simulink model "vrm_plus_ff_return_backup"  (R2013a)
settings: Solver=ode4  SolverMode=SingleTasking  StartTime=0.0  StopTime=inf  FixedStep=0.0005  RelTol=1e-3
StartFcn:
  |  warndlg('Dexterit-E models cannot run under simulation. Please compile your model and run it from within Dexterit-E.');set_param(bdroot,'SimulationCommand','stop')
model workspace (MAT data in the model file):
  BKIN_STEP_TIME = 0.0005
  col_x = 1
  col_y = 2
  E_TARGET_ON = 3
  E_HOLD_AT_TARGET = 5
  LOGICAL_RADIUS = 4
  START_TARGET_COL = 1
  END_TARGET_COL = 2
  ROTATION_CENTER = 3
  WAIT_AT_1stTARGET_COL = 4
  MAXREACHTIME_COL = 5
  WAIT_AT_2ndTARGET_COL = 6
  ROTATION_TYPE = 8
  ROTATION = 9
  DELAY_POSTTRIAL_COL = 7
  E_STAY_CENTER = 2
  VISUAL_RADIUS = 3
  COLOR = 5
  ALTCOLOR = 6
  A_VISC = 1
  B_VISC = 2
  C_VISC = 3
  D_VISC = 4
  LOAD = 10
  TRAJ_DURATION_COL = 11
undefined symbols (not defined in the file or in its folder): slselsubs
libraries: General x3, KINARM_EP_loads x3, Video x3, KINARM_general x1, simulink x1, KINARM_loads x1
(part 1 of 2)
CloseFcn:
  | rtwprivate ssgencode ModelCloseRequest b2lab2d
settings Model: ModifiedComment=chris -- Wed Feb 16 09:18:30 2005 -- Version 1.1384  ModifiedHistory=Feb 16/05 - Add error repeat, add offset ramp  ExtModeArmWhenConnect=off  ExtModeLogAll=off  BufferReuse=off  Creator=Chris Grebeldinger  LastModifiedBy=BKIN TECHNOLOGIES
settings DataIOCC: LimitDataPoints=off  SignalLoggingSaveFormat=ModelDataLogs  SaveOutput=off  SaveTime=off  SignalLoggingName=sigsOut
settings OptimizationCC: BlockReduction=off  BooleanDataType=off  OptimizeBlockIOStorage=off  BufferReuse=off  ExpressionFolding=off  ExpressionDepthLimit=2147483647  FoldNonRolledExpr=off  LocalBlockOutputs=off  InitFltsAndDblsToZero=on
settings DebuggingCC: SaveWithParameterizedLinksMsg=none  SignalResolutionControl=TryResolveAllWithWarning  SolverPrmCheckMsg=none  MultiTaskDSMMsg=warning  MultiTaskCondExecSysMsg=none  FcnCallInpInsideContextMsg=UseLocalSettings  StrictBusMsg=None
settings HardwareCC: ProdIntDivRoundTo=Zero  ProdEndianess=LittleEndian  ProdHWDeviceType=Generic->32-bit x86 compatible  TargetHWDeviceType=32-bit Generic
settings SFSimCC: SimParseCustomCode=off
settings RTWCC: SystemTargetFile=xpctarget.tlc  TemplateMakefile=xpc_default_tmf  Description=xPC Target  ProcessScript=xpctarget_make_rtw_hook  IncludeERTFirstTime=on  RTWCompilerOptimization=On
settings CodeAppCC: MaxIdLength=63
settings xpcTargetCC: TargetFcnLib=ansi_tfl_tmw.mat  CodeReplacementLibrary=XPC_BLAS  ParMdlRefBuildCompliant=on  ConcurrentExecutionCompliant=on  CombineSignalStateStructs=off  MATLABClassNameForMDSCustomization=xpcAperiodicCustomization  GRTInterface=on  GenerateAllocFcn=off  xPCTaskExecutionProfile=off  xPCRL32EventNumber=5000  xPCisDownloadable=off  xPCLoadParamSetFile=off  xPCConcurrentTasks=off  xPCEnableSFAnimation=off

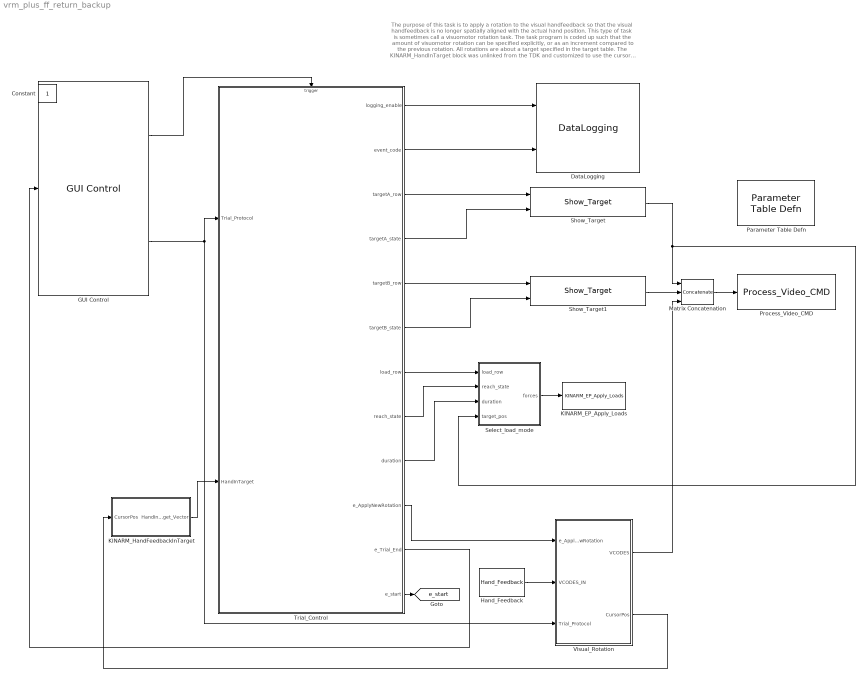
== system vrm_plus_ff_return_backup ==
  note: The purpose of this task is to apply a rotation to the visual handfeedback so that the visual handfeedback is no longer spatially aligned with the actual hand position.
      | This type of task is sometimes call a visuomotor rotation task.
      | The task program is coded up such that the amount of visuomotor rotation can be specified explicitly, or as an increment compared to the previous rotation.
      | All rotations are about a target specified in the target table.
      |
      | The KINARM_HandInTarget block was unlinked from the TDK and customized to use the cursor position as hand feedback input, rather than the KINARM robot's actual location.
  DataLogging : General/DataLogging  log_event_codes=on  log_analog_inputs=off
      link override Poll KINARM/EPTorqueCMD: GotoTag=KINARMEPTorqueCMD
  GUI Control : General/GUI Control  target_type_str=Circle  Target_Type=1  XYcols=[1 2]  Vcols=3  Lcols=4  indices_padding=[0 0 0 0;0 0 0 0]  task_version=1.0  show_repeat_trial_flag=off
  Hand_Feedback : KINARM_general/Hand_Feedback  feedback_cntl_src=none
  KINARM_EP_Apply_Loads : KINARM_EP_loads/KINARM_EP_Apply_Loads  up_duration=1500  down_duration=1500  max_force=60
  KINARM_HandFeedbackInTarget : Subsystem  AncestorBlock=KINARM_general/KINARM_HandInTarget  mask(KINARM_HandInTarget){use_dominant_hand=on, target_type=Circle, num_states=1, attribcol1=4, attribcol2=3, attribcol3=3, attribcol4=3}
      mask prompts: use_dominant_hand "Dominant Hand?"; target_type "Type of Target"; num_states "Number of Target States"; attribcol1 "State 1 Target Table Column(s)"; attribcol2 "State 2 Target Table Column(s)"; attribcol3 "State 3 Target Table Column(s)"; attribcol4 "State 4 Target Table Column(s)"
      mask help: This block returns a vector or array corresponding to the Target_Table rows indicating whether the specified hand is in (=1) or out (=0) of each of the targets.
      mask init:
      | num_states=str2num(get_param(gcb, 'num_states'));
      | columntext='(columns: ';
      | 
      | for i=1:num_states
      | 	varname=['attribcol' num2str(i)];
      | 	if i>1
      | 		columntext=[columntext, '; '];
      | 	end
      | 	columntext=[columntext, get_param(gcb, varname)];
      | end
      | columntext=strvcat([columntext ')'],' ', ' ');
      | 
      | output_block=char(find_system(gcb,'LookUnderMasks','all','FollowLinks','on','SearchDepth',1,'BlockType','Outport'));
      | outputname=get_param(output_block,'Name');
      | 
      | % Select only the desired states for output. The output port is also renamed to reflect 
      | % whether the output is a vector (in the case of a single state) or an array (of vectors, 
      | % one for each of multiple states).
      | if num_states == 1
      | 	set_param([gcb '/Selected States'], 'Value', '[1]');
      | 	set_param(output_block, 'Name', 'HandInTarget_Vector');
      | elseif num_states == 2
      | 	set_param([gcb '/Selected States'], 'Value', '[1,2]');
      | 	set_param(output_block, 'Name', 'HandInTarget_Array');
      | elseif num_states == 3
      | 	set_param([gcb '/Selected States'], 'Value', '[1,2,3]');
      | 	set_param(output_block, 'Name', 'HandInTarget_Array');
      | else
      | 	set_param([gcb '/Selected States'], 'Value', '[1,2,3,4]');
      | 	set_param(output_block, 'Name', 'HandInTarget_Array');
      | end
      mask Help:
      | Used to determine if the hand (finger-tip) is in any of the targets in the Target_Table.
      | <P>
      | <B><I>Use of this block requires that the DataLogging block (General library) be set to log KINARM data.</I></B>
      | 
      | <H2>Library </H2>
      | KINARM_general (sub-library)
      | 
      | <H2>Description </H2>
      | This block returns a vector or array corresponding to the Target_Table rows indicating whether the specified hand (i.e. finger-tip) is in or out of each of the targets.  Each element in the output vector or output array will be either a 0 (hand not in target) or a 1 (hand in target).
      | <P>
      | A vector is returned if only one target state is specified in each target row (see Parameters and Dialog Box), with each index of the vector corresponding to a row in the target table.  An array is returned if more than one target state is specified in a target row, with each row of the array corresponding to a target row and each column corresponding to the nth target state specified in each target row.
      | <P>
      | The output vector or array is typically used by a stateflow chart to affect behavior of the system.  Because this block returns hand-in-target information for all targets in the target table, multiple targets can be monitored at once (i.e. the stateflow chart could have certain transitions that occur if the hand is in one target and other transitions if it is in a different target).  Likewise, because this block returns hand-in-target information for multiple states of a single target, those multiple states can be monitored simultaneously.
      | <P>
      | Because the KINARM_HandInTarget block returns information for only one hand, two copies of this block are required if information for both hands is desired.
      | <P>
      | 
      | <H2>Parameters and Dialog Box</H2>
      | <B>Dominant Hand?:</B> this box determines which hand is used by this block : dominant hand position (checked box) or the non-dominant hand position (unchecked box).  (Note: if the end-user wants to know about both the dominant hand and the non-dominant hand, then 2 separate copies of this block are requried, one for each hand.)
      | <P>
      | <B>Type of Target:</B> Enter the type of target specified in the target table:
      | <P>
      | <B>Number of Target States:</B> Enter the number of target states specified in each target row.  Up to four target states are allowed per target row.
      | <P>
      | <B>State <n> Target Table Columns:</B> Enter the columns in the Target Table that specify the relevant target attributes.  Do this for each target state.
      | For a circle, enter the columns corresponding to logical radius (e.g. 4)
      | <BR>For an ellipse, enter the columns corresponding to major radius, minor radius, rotation angle (e.g. [4, 5, 6]).
      | <BR>For a rectangle, enter the columns corresponding to length, height, and rotation angle (e.g. [4, 5, 6]).
      | <BR>For a line, enter the columns corresponding to stroke width, endpoint in x, and endpoint in y (e.g. [3, 4, 5]).
      | <BR>For a triangle, enter the columns corresponding to length, height, peak offset, and rotation angle (e.g. [4, 5, 6, 7]).
      | 
      | <H2>Examples</H2>
      | <B>Example 1.</B>  Suppose a target row will be used to define 1 state for a circle type target and the radius of the visual target is the same radius to be used for determination of hand-in-target.  The related Target Table column is: column 6 = radius.  For this example, "State 1 Target Table Columns" would equal [6].
      | <P>
      | 
      | <B>Example 2.</B>  Suppose a target row will be used to define 1 state for a circle type target, but the radius of the visual target will be different than the radius to be used for determination of hand-in-target.  This option allows independent control over the size of the visual target versus the accuracy needed to be considered "in the target".  The related Target Table columns are: column 6 = radius1 (i.e. radius to target to be drawn); column 7 = radius2 (i.e. radius to be used for hand-in-target) .  For this example, "State 1 Target Table Columns" would equal [7].
      | <P>
      | <B>Example 3.</B>  Suppose a target row will be used to define 2 states for a circle type target, where the radius of the visual target will be a constant, but depending on the state of the system, one of 2 other and different radii will be used for determination of hand-in-target.  The related Target Table columns are: column 6 = radius1 (i.e. radius to target to be drawn); column 7 = radius2 (i.e. radius to be used for hand-in-target for state 1); column 8 = radius3 (i.e. radius to be used for hand-in-target for state 2).  For this example, "State 1 Target Table Columns" would equal [7], while "State 2 Target Table Columns" would equal [8].
      | <P>
      | 
      | <H2>Related Blocks </H2>
      | DataLogging
      mask TypeOptions target_type: Circle | Ellipse | Rectangle | Line | Triangle
      mask Callback target_type:
      | target_type=get_param(gcb, 'target_type');
      | attribcol1=[str2num(get_param(gcb, 'attribcol1')) 0 0 0 0 0 0];
      | attribcol2=[str2num(get_param(gcb, 'attribcol2')) 0 0 0 0 0 0];
      | attribcol3=[str2num(get_param(gcb, 'attribcol3')) 0 0 0 0 0 0];
      | attribcol4=[str2num(get_param(gcb, 'attribcol4')) 0 0 0 0 0 0];
      | switch target_type(1:3)
      | 	case 'Cir'
      | 		numcol=1;
      | 	case 'Ell'
      | 		numcol=3;
      |     case 'Rec'
      |         numcol=3;
      |     case 'Lin'
      |         numcol=3;
      |     case 'Tri'
      |         numcol=4;
      | 	otherwise
      | 		numcol=1;
      | end
      | if numcol==1
      | 	set_param(gcb, 'attribcol1', num2str(attribcol1(1)));
      | 	set_param(gcb, 'attribcol2', num2str(attribcol2(1)));
      | 	set_param(gcb, 'attribcol3', num2str(attribcol3(1)));
      | 	set_param(gcb, 'attribcol4', num2str(attribcol4(1)));
      | else
      | 	set_param(gcb, 'attribcol1', ['[' num2str(attribcol1(1:numcol)) ']']);
      | 	set_param(gcb, 'attribcol2', ['[' num2str(attribcol2(1:numcol)) ']']);
      | 	set_param(gcb, 'attribcol3', ['[' num2str(attribcol3(1:numcol)) ']']);
      | 	set_param(gcb, 'attribcol4', ['[' num2str(attribcol4(1:numcol)) ']']);
      | end
      mask TypeOptions num_states: 1 | 2 | 3 | 4
      mask Callback num_states:
      | num_states = str2num(get_param(gcb, 'num_states'));
      | vis = get_param(gcb, 'MaskVisibilities');
      | 
      | % Select only the desired states for output. The output port is also renamed to reflect
      | % whether the output is a vector (in the case of a single state) or an array (of vectors,
      | % one for each of multiple states).
      | output_block=char(find_system(gcb, 'LookUnderMasks', 'all', 'FollowLinks', 'on', 'SearchDepth', 1, 'BlockType', 'Outport'));
      | 
      | if num_states == 1
      | 	set_param([gcb '/Selected States'], 'Value', '[1]');
      | 	set_param(output_block, 'Name', 'HandInTarget_Vector');
      | 	vis{5} = 'off';
      | 	vis{6} = 'off';
      | 	vis{7} = 'off';
      | elseif num_states == 2
      | 	set_param([gcb '/Selected States'], 'Value', '[1,2]');
      | 	set_param(output_block, 'Name', 'HandInTarget_Array');
      | 	vis{5} = 'on';
      | 	vis{6} = 'off';
      | 	vis{7} = 'off';
      | elseif num_states == 3
      | 	set_param([gcb '/Selected States'], 'Value', '[1,2,3]');
      | 	set_param(output_block, 'Name','HandInTarget_Array');
      | 	vis{5} = 'on';
      | 	vis{6} = 'on';
      | 	vis{7} = 'off';
      | else
      | 	set_param([gcb '/Selected States'], 'Value', '[1,2,3,4]');
      | 	set_param(output_block, 'Name', 'HandInTarget_Array');
      | 	vis{5} = 'on';
      | 	vis{6} = 'on';
      | 	vis{7} = 'on';
      | end
      | set_param(gcb, 'MaskVisibilities', vis);
      | 
      | target_type=get_param(gcb, 'target_type');
      | attribcol1=[str2num(get_param(gcb, 'attribcol1')) 0 0 0 0 0 0];
      | attribcol2=[str2num(get_param(gcb, 'attribcol2')) 0 0 0 0 0 0];
      | attribcol3=[str2num(get_param(gcb, 'attribcol3')) 0 0 0 0 0 0];
      | attribcol4=[str2num(get_param(gcb, 'attribcol4')) 0 0 0 0 0 0];
      | switch target_type(1:3)
      | 	case 'Cir'
      | 		numcol=1;
      | 	case 'Ell'
      | 		numcol=3;
      |     case 'Rec'
      |         numcol=3;
      |     case 'Lin'
      |         numcol=3;
      |     case 'Tri'
      |         numcol=4;
      | 	otherwise
      | 		numcol=1;
      | end
      | if numcol==1
      | 	set_param(gcb, 'attribcol1', num2str(attribcol1(1)));
      | 	set_param(gcb, 'attribcol2', num2str(attribcol2(1)));
      | 	set_param(gcb, 'attribcol3', num2str(attribcol3(1)));
      | 	set_param(gcb, 'attribcol4', num2str(attribcol4(1)));
      | else
      | 	set_param(gcb, 'attribcol1', ['[' num2str(attribcol1(1:numcol)) ']']);
      | 	set_param(gcb, 'attribcol2', ['[' num2str(attribcol2(1:numcol)) ']']);
      | 	set_param(gcb, 'attribcol3', ['[' num2str(attribcol3(1:numcol)) ']']);
      | 	set_param(gcb, 'attribcol4', ['[' num2str(attribcol4(1:numcol)) ']']);
      | end
      mask Callback attribcol1:
      | target_type=get_param(gcb, 'target_type');
      | attribcol1=[str2num(get_param(gcb, 'attribcol1')) 0 0 0 0 0 0];
      | attribcol2=[str2num(get_param(gcb, 'attribcol2')) 0 0 0 0 0 0];
      | attribcol3=[str2num(get_param(gcb, 'attribcol3')) 0 0 0 0 0 0];
      | attribcol4=[str2num(get_param(gcb, 'attribcol4')) 0 0 0 0 0 0];
      | switch target_type(1:3)
      | 	case 'Cir'
      | 		numcol=1;
      | 	case 'Ell'
      | 		numcol=3;
      |     case 'Rec'
      |         numcol=3;
      |     case 'Lin'
      |         numcol=3;
      |     case 'Tri'
      |         numcol=4;
      | 	otherwise
      | 		numcol=1;
      | end
      | if numcol==1
      | 	set_param(gcb, 'attribcol1', num2str(attribcol1(1)));
      | 	set_param(gcb, 'attribcol2', num2str(attribcol2(1)));
      | 	set_param(gcb, 'attribcol3', num2str(attribcol3(1)));
      | 	set_param(gcb, 'attribcol4', num2str(attribcol4(1)));
      | else
      | 	set_param(gcb, 'attribcol1', ['[' num2str(attribcol1(1:numcol)) ']']);
      | 	set_param(gcb, 'attribcol2', ['[' num2str(attribcol2(1:numcol)) ']']);
      | 	set_param(gcb, 'attribcol3', ['[' num2str(attribcol3(1:numcol)) ']']);
      | 	set_param(gcb, 'attribcol4', ['[' num2str(attribcol4(1:numcol)) ']']);
      | end
      mask Callback attribcol2:
      | target_type=get_param(gcb, 'target_type');
      | attribcol1=[str2num(get_param(gcb, 'attribcol1')) 0 0 0 0 0 0];
      | attribcol2=[str2num(get_param(gcb, 'attribcol2')) 0 0 0 0 0 0];
      | attribcol3=[str2num(get_param(gcb, 'attribcol3')) 0 0 0 0 0 0];
      | attribcol4=[str2num(get_param(gcb, 'attribcol4')) 0 0 0 0 0 0];
      | switch target_type(1:3)
      | 	case 'Cir'
      | 		numcol=1;
      | 	case 'Ell'
      | 		numcol=3;
      |     case 'Rec'
      |         numcol=3;
      |     case 'Lin'
      |         numcol=3;
      |     case 'Tri'
      |         numcol=4;
      | 	otherwise
      | 		numcol=1;
      | end
      | if numcol==1
      | 	set_param(gcb, 'attribcol1', num2str(attribcol1(1)));
      | 	set_param(gcb, 'attribcol2', num2str(attribcol2(1)));
      | 	set_param(gcb, 'attribcol3', num2str(attribcol3(1)));
      | 	set_param(gcb, 'attribcol4', num2str(attribcol4(1)));
      | else
      | 	set_param(gcb, 'attribcol1', ['[' num2str(attribcol1(1:numcol)) ']']);
      | 	set_param(gcb, 'attribcol2', ['[' num2str(attribcol2(1:numcol)) ']']);
      | 	set_param(gcb, 'attribcol3', ['[' num2str(attribcol3(1:numcol)) ']']);
      | 	set_param(gcb, 'attribcol4', ['[' num2str(attribcol4(1:numcol)) ']']);
      | end
      mask Callback attribcol3:
      | target_type=get_param(gcb, 'target_type');
      | attribcol1=[str2num(get_param(gcb, 'attribcol1')) 0 0 0 0 0 0];
      | attribcol2=[str2num(get_param(gcb, 'attribcol2')) 0 0 0 0 0 0];
      | attribcol3=[str2num(get_param(gcb, 'attribcol3')) 0 0 0 0 0 0];
      | attribcol4=[str2num(get_param(gcb, 'attribcol4')) 0 0 0 0 0 0];
      | switch target_type(1:3)
      | 	case 'Cir'
      | 		numcol=1;
      | 	case 'Ell'
      | 		numcol=3;
      |     case 'Rec'
      |         numcol=3;
      |     case 'Lin'
      |         numcol=3;
      |     case 'Tri'
      |         numcol=4;
      | 	otherwise
      | 		numcol=1;
      | end
      | if numcol==1
      | 	set_param(gcb, 'attribcol1', num2str(attribcol1(1)));
      | 	set_param(gcb, 'attribcol2', num2str(attribcol2(1)));
      | 	set_param(gcb, 'attribcol3', num2str(attribcol3(1)));
      | 	set_param(gcb, 'attribcol4', num2str(attribcol4(1)));
      | else
      | 	set_param(gcb, 'attribcol1', ['[' num2str(attribcol1(1:numcol)) ']']);
      | 	set_param(gcb, 'attribcol2', ['[' num2str(attribcol2(1:numcol)) ']']);
      | 	set_param(gcb, 'attribcol3', ['[' num2str(attribcol3(1:numcol)) ']']);
      | 	set_param(gcb, 'attribcol4', ['[' num2str(attribcol4(1:numcol)) ']']);
      | end
      mask Callback attribcol4:
      | target_type=get_param(gcb, 'target_type');
      | attribcol1=[str2num(get_param(gcb, 'attribcol1')) 0 0 0 0 0 0];
      | attribcol2=[str2num(get_param(gcb, 'attribcol2')) 0 0 0 0 0 0];
      | attribcol3=[str2num(get_param(gcb, 'attribcol3')) 0 0 0 0 0 0];
      | attribcol4=[str2num(get_param(gcb, 'attribcol4')) 0 0 0 0 0 0];
      | switch target_type(1:3)
      | 	case 'Cir'
      | 		numcol=1;
      | 	case 'Ell'
      | 		numcol=3;
      |     case 'Rec'
      |         numcol=3;
      |     case 'Lin'
      |         numcol=3;
      |     case 'Tri'
      |         numcol=4;
      | 	otherwise
      | 		numcol=1;
      | end
      | if numcol==1
      | 	set_param(gcb, 'attribcol1', num2str(attribcol1(1)));
      | 	set_param(gcb, 'attribcol2', num2str(attribcol2(1)));
      | 	set_param(gcb, 'attribcol3', num2str(attribcol3(1)));
      | 	set_param(gcb, 'attribcol4', num2str(attribcol4(1)));
      | else
      | 	set_param(gcb, 'attribcol1', ['[' num2str(attribcol1(1:numcol)) ']']);
      | 	set_param(gcb, 'attribcol2', ['[' num2str(attribcol2(1:numcol)) ']']);
      | 	set_param(gcb, 'attribcol3', ['[' num2str(attribcol3(1:numcol)) ']']);
      | 	set_param(gcb, 'attribcol4', ['[' num2str(attribcol4(1:numcol)) ']']);
      | end
      mask Display:
      | disp(columntext)
      | port_label('output',1,outputname)
  Matrix Concatenation : Concatenate  NumInputs=3  Mode=Multidimensional array
  Parameter Table Defn : General/Parameter Table Defn  ShowInLibBrowser=0
  Process_Video_CMD : Video/Process_Video_CMD
  Select_load_mode : Subsystem
  Show_Target : Video/Show_Target  target_type=Circle  num_states=2  attribcol1=[COLOR 0 0 VISUAL_RADIUS]  attribcol2=[ALTCOLOR 0 0 VISUAL_RADIUS]  attribcol3=[0 0 0 0]  attribcol4=[0 0 0 0]  attribcol5=[0 0 24 0]  stateindices_padding=[0 0 0 0 0 0 0;0 0 0 0 0 0 0;0 0 0 0 0 0 0;0 0 0 0 0 0 0;0 0 0 0 0 0 0]  source=dialog  opacity=100  target_display=Both subject and operator displays  num_col=4
  Show_Target1 : Video/Show_Target  target_type=Circle  num_states=2  attribcol1=[COLOR 0 0 VISUAL_RADIUS]  attribcol2=[ALTCOLOR 0 0 VISUAL_RADIUS]  attribcol3=[0 0 0 0]  attribcol4=[0 0 0 0]  attribcol5=[0 0 24 0]  stateindices_padding=[0 0 0 0 0 0 0;0 0 0 0 0 0 0;0 0 0 0 0 0 0;0 0 0 0 0 0 0;0 0 0 0 0 0 0]  source=dialog  opacity=100  target_display=Both subject and operator displays  num_col=4
  Trial_Control : Stateflow chart  TreatAsAtomicUnit=on
  Visual_Rotation : Subsystem
  Constant : Constant  IOType=siggen
  tag scope: e_start=global
  wires:
  GUI Control/2 -> Visual_Rotation/3(Trial_Protocol), Trial_Control/1(Trial_Protocol)
  Trial_Control/11(e_Trial_End) -> GUI Control/1
  GUI Control/1 -> Trial_Control/Trigger
  Trial_Control/4(targetA_state) -> Show_Target/2
  Trial_Control/3(targetA_row) -> Show_Target/1
  Show_Target1/1 -> Matrix Concatenation/2
  Trial_Control/5(targetB_row) -> Show_Target1/1
  Trial_Control/6(targetB_state) -> Show_Target1/2
  Trial_Control/2(event_code) -> DataLogging/2
  Matrix Concatenation/1 -> Process_Video_CMD/1
  Hand_Feedback/1 -> Visual_Rotation/2(VCODES_IN)
  Visual_Rotation/2(CursorPos) -> KINARM_HandFeedbackInTarget/1(CursorPos)
  KINARM_HandFeedbackInTarget/1(HandInTarget_Vector) -> Trial_Control/2(HandInTarget)
  Trial_Control/10(e_ApplyNewRotation) -> Visual_Rotation/1(e_ApplyNewRotation)
  Visual_Rotation/1(VCODES) -> Matrix Concatenation/3
  Trial_Control/1(logging_enable) -> DataLogging/1
  Select_load_mode/1(forces) -> KINARM_EP_Apply_Loads/1
  Trial_Control/7(load_row) -> Select_load_mode/1(load_row)
  Trial_Control/8(reach_state) -> Select_load_mode/2(reach_state)
  Trial_Control/12(e_start) -> [e_start]
  Trial_Control/9(duration) -> Select_load_mode/3(duration)
  Show_Target/1 -> Matrix Concatenation/1, Select_load_mode/4(target_pos)

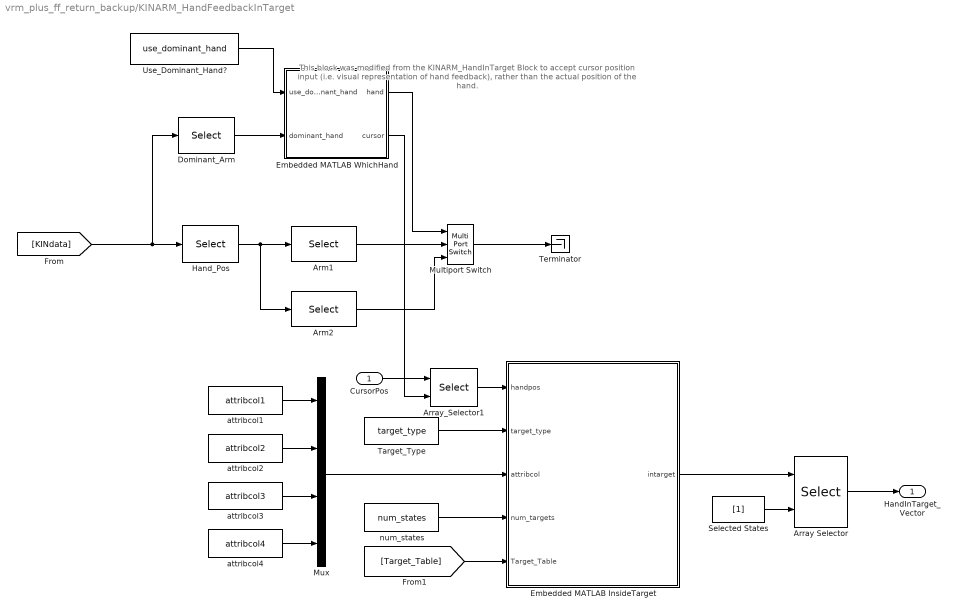
== system vrm_plus_ff_return_backup/KINARM_HandFeedbackInTarget ==
  note: This block was modified from the KINARM_HandInTarget Block to accept cursor position input (i.e. visual
      | representation of hand feedback), rather than the actual position of the hand.
  CursorPos : Inport
  Arm1 : Selector  NumberOfDimensions=2  InputPortWidth=3  IndexOptions=Index vector (dialog),Select all  Indices=1,-1  OutputSizes=slselsubs([(-2),(-2)],1),slselsubs([(-2),(-2)],2)
  Arm2 : Selector  NumberOfDimensions=2  InputPortWidth=3  IndexOptions=Index vector (dialog),Select all  Indices=2,-1  OutputSizes=slselsubs([(-2),(-2)],1),slselsubs([(-2),(-2)],2)
  Array Selector : Selector  NumberOfDimensions=2  InputPortWidth=3  IndexOptions=Select all,Index vector (port)  Indices=-1,1  OutputSizes=slselsubs([(-2),(-2)],1),slselsubs([(-2),(-2)],2)
  Array_Selector1 : Selector  NumberOfDimensions=2  InputPortWidth=3  IndexOptions=Index vector (port),Select all  Indices=-1,1  OutputSizes=1
  Dominant_Arm : Selector  NumberOfDimensions=2  InputPortWidth=3  IndexOptions=Index vector (dialog),Index vector (dialog)  Indices=[3],[1]  OutputSizes=slselsubs([(-2),(-2)],1),slselsubs([(-2),(-2)],2)
  Embedded MATLAB InsideTarget : MATLAB Function  TreatAsAtomicUnit=on
  Embedded MATLAB WhichHand : MATLAB Function  TreatAsAtomicUnit=on
  Hand_Pos : Selector  NumberOfDimensions=2  InputPortWidth=3  IndexOptions=Select all,Index vector (dialog)  Indices=-1,[23,24]  OutputSizes=slselsubs([(-2),(-2)],1),slselsubs([(-2),(-2)],2)
  Multiport Switch : MultiPortSwitch  Inputs=2
  Mux : Mux
  Selected States : Constant  Value=[1]
  Target_Type : Constant  Value=target_type
  Terminator : Terminator
  Use_Dominant_Hand? : Constant  Value=use_dominant_hand
  attribcol1 : Constant  Value=attribcol1
  attribcol2 : Constant  Value=attribcol2
  attribcol3 : Constant  Value=attribcol3
  attribcol4 : Constant  Value=attribcol4
  num_states : Constant  Value=num_states
  HandInTarget_Vector : Outport
  wires:
  Selected States/1 -> Array Selector/2
  num_states/1 -> Embedded MATLAB InsideTarget/4(num_targets)
  Mux/1 -> Embedded MATLAB InsideTarget/3(attribcol)
  attribcol4/1 -> Mux/4
  attribcol3/1 -> Mux/3
  attribcol2/1 -> Mux/2
  attribcol1/1 -> Mux/1
  Use_Dominant_Hand?/1 -> Embedded MATLAB WhichHand/1(use_dominant_hand)
  Embedded MATLAB WhichHand/1(hand) -> Multiport Switch/1
  Target_Type/1 -> Embedded MATLAB InsideTarget/2(target_type)
  Array Selector/1 -> HandInTarget_Vector/1
  [Target_Table] -> Embedded MATLAB InsideTarget/5(Target_Table)
  Embedded MATLAB InsideTarget/1(intarget) -> Array Selector/1
  Multiport Switch/1 -> Terminator/1
  Arm2/1 -> Multiport Switch/3
  Arm1/1 -> Multiport Switch/2
  Dominant_Arm/1 -> Embedded MATLAB WhichHand/2(dominant_hand)
  Hand_Pos/1 -> Arm2/1, Arm1/1
  [KINdata] -> Dominant_Arm/1, Hand_Pos/1
  CursorPos/1 -> Array_Selector1/1
  Array_Selector1/1 -> Embedded MATLAB InsideTarget/1(handpos)
  Embedded MATLAB WhichHand/2(cursor) -> Array_Selector1/2

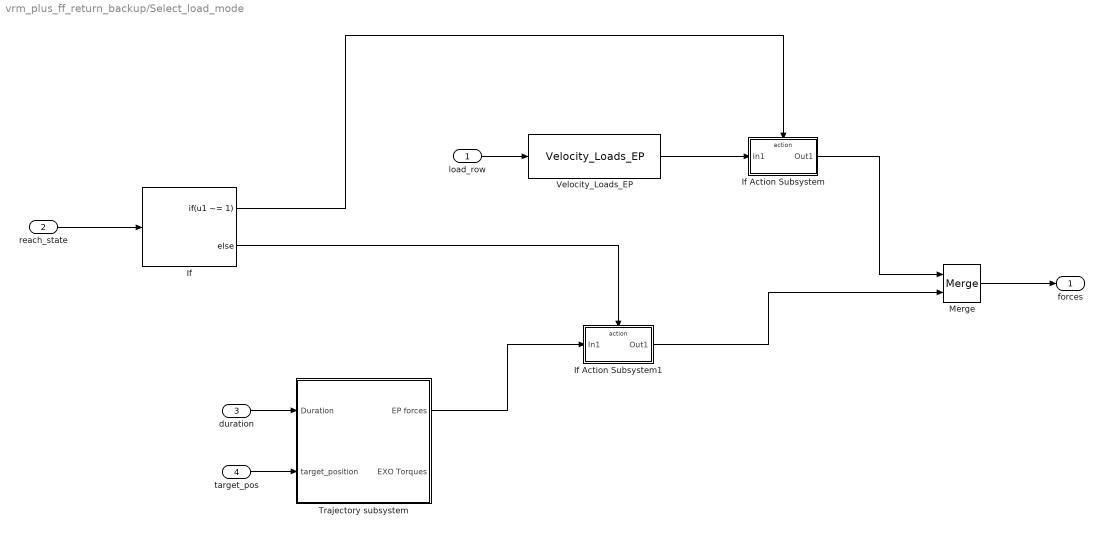
== system vrm_plus_ff_return_backup/Select_load_mode ==
  load_row : Inport
  reach_state : Inport  Port=2
  duration : Inport  Port=3
  target_pos : Inport  Port=4
  If : If  IfExpression=u1 ~= 1
  If Action Subsystem : Subsystem  TreatAsAtomicUnit=on
  If Action Subsystem1 : Subsystem  TreatAsAtomicUnit=on
  Merge : Merge
  Trajectory subsystem : Subsystem
  Velocity_Loads_EP : KINARM_EP_loads/Velocity_Loads_EP  use_dom_hand=on  loadcol=[A_VISC B_VISC C_VISC D_VISC]  source=dialog  scaling=1  stability=on
  forces : Outport
  wires:
  If/1 -> If Action Subsystem/Action
  If/2 -> If Action Subsystem1/Action
  If Action Subsystem1/1(Out1) -> Merge/2
  reach_state/1 -> If/1
  load_row/1 -> Velocity_Loads_EP/1
  duration/1 -> Trajectory subsystem/1(Duration)
  target_pos/1 -> Trajectory subsystem/2(target_position)
  Velocity_Loads_EP/1 -> If Action Subsystem/1(In1)
  If Action Subsystem/1(Out1) -> Merge/1
  Trajectory subsystem/1(EP forces) -> If Action Subsystem1/1(In1)
  Merge/1 -> forces/1

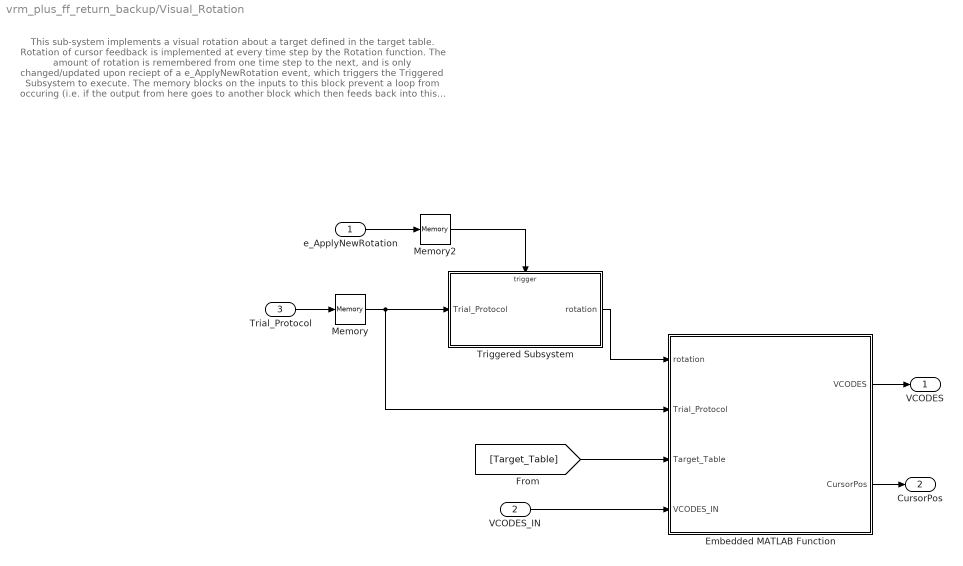
== system vrm_plus_ff_return_backup/Visual_Rotation ==
  note: This sub-system implements a visual rotation about a target defined in the target table.
      |
      | Rotation of cursor feedback is implemented at every time step by the Rotation function.
      | The amount of rotation is remembered from one time step to the next, and is only changed/updated
      | upon reciept of a e_ApplyNewRotation event, which triggers the Triggered Subsystem to execute.
      |
      | The memory blocks on the inputs to this block prevent a loop from occuring (i.e. if the output from here goes to
      | another block which then feeds back into this block, which forms a loop, which needs to be broken by the Memory block).
  e_ApplyNewRotation : Inport
  VCODES_IN : Inport  Port=2
  Trial_Protocol : Inport  Port=3
  Embedded MATLAB Function : MATLAB Function  TreatAsAtomicUnit=on
  Memory : Memory  InheritSampleTime=on
  Memory2 : Memory  InheritSampleTime=on
  Triggered Subsystem : Subsystem  TreatAsAtomicUnit=on
  VCODES : Outport
  CursorPos : Outport  Port=2
  wires:
  Trial_Protocol/1 -> Memory/1
  Embedded MATLAB Function/1(VCODES) -> VCODES/1
  VCODES_IN/1 -> Embedded MATLAB Function/4(VCODES_IN)
  Embedded MATLAB Function/2(CursorPos) -> CursorPos/1
  Memory/1 -> Triggered Subsystem/1(Trial_Protocol), Embedded MATLAB Function/2(Trial_Protocol)
  e_ApplyNewRotation/1 -> Memory2/1
  Triggered Subsystem/1(rotation) -> Embedded MATLAB Function/1(rotation)
  [Target_Table] -> Embedded MATLAB Function/3(Target_Table)
  Memory2/1 -> Triggered Subsystem/Trigger

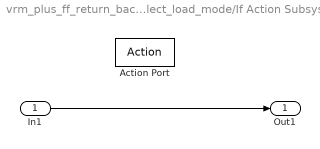
== system vrm_plus_ff_return_backup/Select_load_mode/If Action Subsystem ==
  In1 : Inport
  Action Port : ActionPort  ActionType=then
  Out1 : Outport
  wires:
  In1/1 -> Out1/1

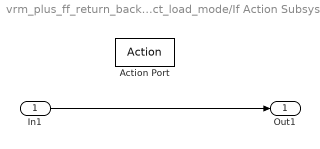
== system vrm_plus_ff_return_backup/Select_load_mode/If Action Subsystem1 ==
  In1 : Inport
  Action Port : ActionPort  ActionType=else
  Out1 : Outport
  wires:
  In1/1 -> Out1/1

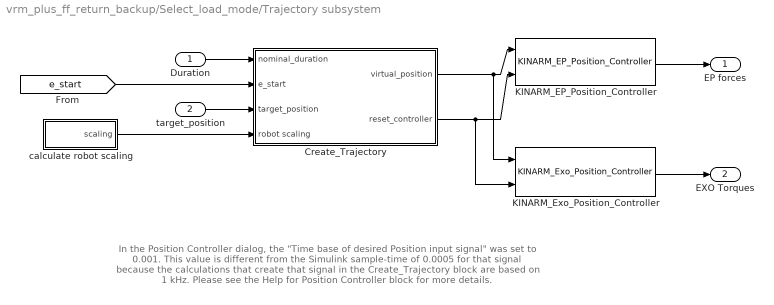
== system vrm_plus_ff_return_backup/Select_load_mode/Trajectory subsystem ==
  note: In the Position Controller dialog, the "Time base of desired Position input signal" was set to 0.001.
      | This value is different from the Simulink sample-time of 0.0005 for that signal because the calculations
      | that create that signal in the Create_Trajectory block are based on 1 kHz. Please see the Help for
      | Position Controller block for more details.
  Duration : Inport
  target_position : Inport  Port=2
  Create_Trajectory : Subsystem
  KINARM_EP_Position_Controller : KINARM_EP_loads/KINARM_EP_Position_Controller  use_dom_hand=on  inertias_for_FF=KINARM End Point robot  gain_choice=Standard Movement  sample_time=0.001
  KINARM_Exo_Position_Controller : KINARM_loads/KINARM_Exo_Position_Controller  use_dom_hand=on  KINARM_Type=Human  inertias_for_FF=KINARM robot  angles_or_XY=End-point (global x/y)  sample_time=0.001
  calculate robot scaling : Subsystem
  EP forces : Outport
  EXO Torques : Outport  Port=2
  wires:
  Create_Trajectory/2(reset_controller) -> KINARM_EP_Position_Controller/2, KINARM_Exo_Position_Controller/2
  Create_Trajectory/1(virtual_position) -> KINARM_EP_Position_Controller/1, KINARM_Exo_Position_Controller/1
  KINARM_EP_Position_Controller/1 -> EP forces/1
  KINARM_Exo_Position_Controller/1 -> EXO Torques/1
  target_position/1 -> Create_Trajectory/3(target_position)
  Duration/1 -> Create_Trajectory/1(nominal_duration)
  [e_start] -> Create_Trajectory/2(e_start)
  calculate robot scaling/1(scaling) -> Create_Trajectory/4(robot scaling)

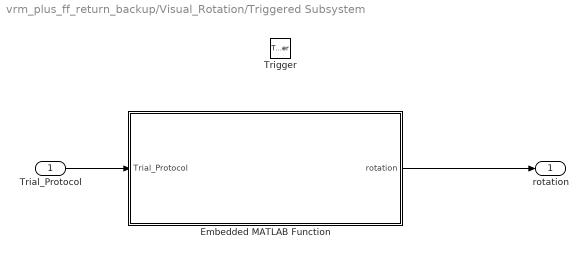
== system vrm_plus_ff_return_backup/Visual_Rotation/Triggered Subsystem ==
  Trial_Protocol : Inport
  Trigger : TriggerPort  TriggerType=either
  Embedded MATLAB Function : MATLAB Function  TreatAsAtomicUnit=on
  rotation : Outport
  wires:
  Trial_Protocol/1 -> Embedded MATLAB Function/1(Trial_Protocol)
  Embedded MATLAB Function/1(rotation) -> rotation/1

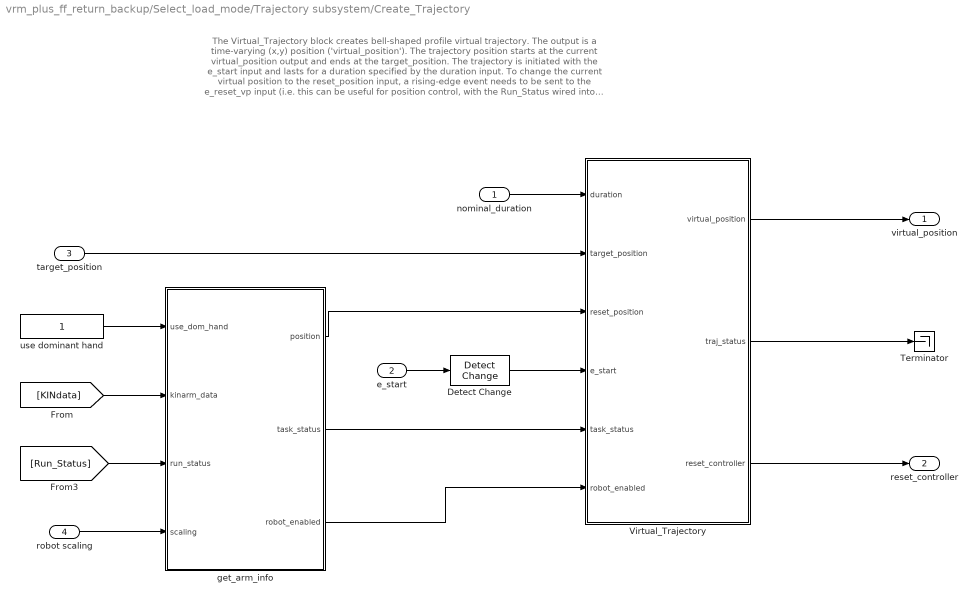
== system vrm_plus_ff_return_backup/Select_load_mode/Trajectory subsystem/Create_Trajectory ==
  note: The Virtual_Trajectory block creates bell-shaped profile virtual trajectory.
      | The output is a time-varying (x,y) position ('virtual_position').
      |
      | The trajectory position starts at the current virtual_position output and ends at the target_position.
      | The trajectory is initiated with the e_start input and lasts for a duration specified by the duration input.
      |
      | To change the current virtual position to the reset_position input, a rising-edge event needs to be sent to the e_reset_vp input
      | (i.e. this can be useful for position control, with the Run_Status wired into the e_reset input).
      | If such an event occurs during a virtual trajectory, the trajectory is halted immediately.
  nominal_duration : Inport
  e_start : Inport  Port=2
  target_position : Inport  Port=3
  robot scaling : Inport  Port=4
  Detect Change : simulink/Logic and Bit Operations/Detect Change  vinit=0  InputProcessing=Inherited  OutDataTypeStr=uint8
  Terminator : Terminator
  Virtual_Trajectory : Subsystem
  get_arm_info : MATLAB Function  TreatAsAtomicUnit=on
  use dominant hand : Constant
  virtual_position : Outport
  reset_controller : Outport  Port=2
  wires:
  Virtual_Trajectory/1(virtual_position) -> virtual_position/1
  nominal_duration/1 -> Virtual_Trajectory/1(duration)
  e_start/1 -> Detect Change/1
  target_position/1 -> Virtual_Trajectory/2(target_position)
  Detect Change/1 -> Virtual_Trajectory/4(e_start)
  use dominant hand/1 -> get_arm_info/1(use_dom_hand)
  [KINdata] -> get_arm_info/2(kinarm_data)
  get_arm_info/1(position) -> Virtual_Trajectory/3(reset_position)
  Virtual_Trajectory/3(reset_controller) -> reset_controller/1
  get_arm_info/2(task_status) -> Virtual_Trajectory/5(task_status)
  get_arm_info/3(robot_enabled) -> Virtual_Trajectory/6(robot_enabled)
  [Run_Status] -> get_arm_info/3(run_status)
  Virtual_Trajectory/2(traj_status) -> Terminator/1
  robot scaling/1 -> get_arm_info/4(scaling)

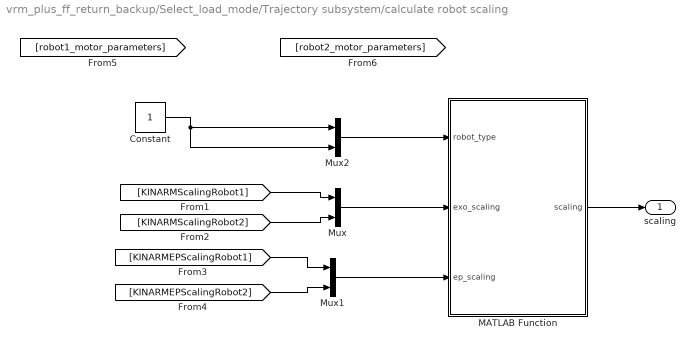
== system vrm_plus_ff_return_backup/Select_load_mode/Trajectory subsystem/calculate robot scaling ==
  Constant : Constant
  MATLAB Function : MATLAB Function  TreatAsAtomicUnit=on
  Mux : Mux  Inputs=2
  Mux1 : Mux  Inputs=2
  Mux2 : Mux  Inputs=2
  scaling : Outport
  wires:
  [KINARMScalingRobot1] -> Mux/1
  [KINARMScalingRobot2] -> Mux/2
  Mux/1 -> MATLAB Function/2(exo_scaling)
  Mux1/1 -> MATLAB Function/3(ep_scaling)
  Mux2/1 -> MATLAB Function/1(robot_type)
  MATLAB Function/1(scaling) -> scaling/1
  [KINARMEPScalingRobot2] -> Mux1/2
  [KINARMEPScalingRobot1] -> Mux1/1
  Constant/1 -> Mux2/1, Mux2/2

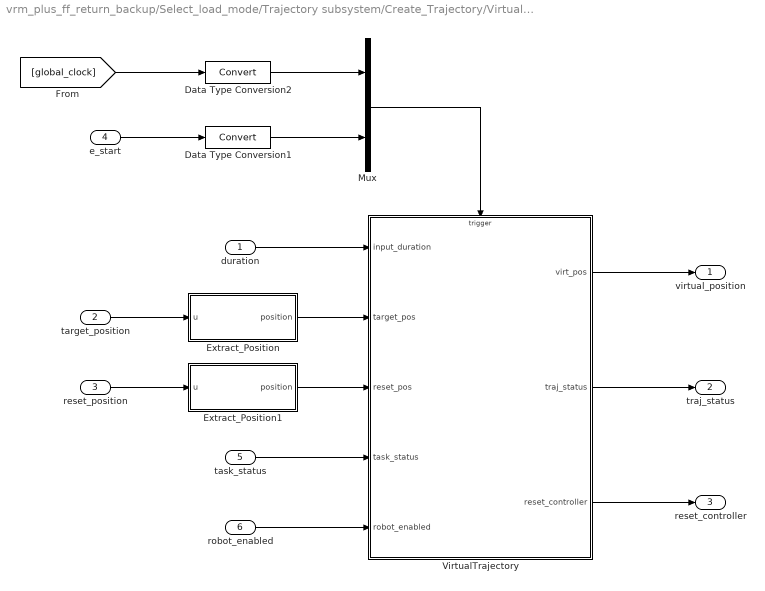
== system vrm_plus_ff_return_backup/Select_load_mode/Trajectory subsystem/Create_Trajectory/Virtual_Trajectory ==
  duration : Inport
  target_position : Inport  Port=2
  reset_position : Inport  Port=3
  e_start : Inport  Port=4
  task_status : Inport  Port=5
  robot_enabled : Inport  Port=6
  Data Type Conversion1 : DataTypeConversion
  Data Type Conversion2 : DataTypeConversion
  Extract_Position : MATLAB Function  TreatAsAtomicUnit=on
  Extract_Position1 : MATLAB Function  TreatAsAtomicUnit=on
  Mux : Mux  Inputs=2
  VirtualTrajectory : Stateflow chart  TreatAsAtomicUnit=on
  virtual_position : Outport
  traj_status : Outport  Port=2
  reset_controller : Outport  Port=3
  wires:
  e_start/1 -> Data Type Conversion1/1
  target_position/1 -> Extract_Position/1(u)
  [global_clock] -> Data Type Conversion2/1
  Mux/1 -> VirtualTrajectory/Trigger
  duration/1 -> VirtualTrajectory/1(input_duration)
  VirtualTrajectory/1(virt_pos) -> virtual_position/1
  Extract_Position/1(position) -> VirtualTrajectory/2(target_pos)
  reset_position/1 -> Extract_Position1/1(u)
  Data Type Conversion2/1 -> Mux/1
  VirtualTrajectory/2(traj_status) -> traj_status/1
  robot_enabled/1 -> VirtualTrajectory/5(robot_enabled)
  task_status/1 -> VirtualTrajectory/4(task_status)
  Data Type Conversion1/1 -> Mux/2
  Extract_Position1/1(position) -> VirtualTrajectory/3(reset_pos)
  VirtualTrajectory/3(reset_controller) -> reset_controller/1

== stateflow chart vrm_plus_ff_return_backup/Trial_Control ==
  settings: sampleTime=0.001
  state Main_Trial
    state FirstTargetOn/
      // Turn on central target, turn on position controller to that target, wait for specified delay or until hand-is-in-target
      targetA_row = Trial_Protocol[START_TARGET_COL];
      targetA_state=1;
      reach_state = 1;
      duration =Trial_Protocol[TRAJ_DURATION_COL];
      e_start;
    state StayAtFirstTarget/
      // change the first target state (e.g. colour), log an event, wait for specified period of time.  Hand must STAY in target for specified time.
      logging_enable = 1;
      event_code=E_STAY_CENTER;
      targetA_state=2;
      tickCount =Trial_Protocol[WAIT_AT_1stTARGET_COL];
      load_row = Trial_Protocol[LOAD];
      reach_state = 2;
    state Show2ndTarget/
      // Turn on second target, log an event, wait until hand-is-in-target or wait for specified delay
      event_code=E_TARGET_ON;
      targetB_row = Trial_Protocol[END_TARGET_COL];
      targetB_state=1;
      tickCount =Trial_Protocol[MAXREACHTIME_COL];
      reach_state = 3;
    state StayAt2ndTarget/
      // change the 2nd target's state, log an event, wait for a specified period of time
      event_code=E_HOLD_AT_TARGET;
      targetB_state=2;
      tickCount =Trial_Protocol[WAIT_AT_2ndTARGET_COL];
      reach_state = 4;
    state EndOfTrial/
      // Wait for a specified period of time,
      tickCount =Trial_Protocol[DELAY_POSTTRIAL_COL];
    FirstTargetOn -> StayAtFirstTarget : [HandInTarget[targetA_row]==1]
    StayAtFirstTarget -> FirstTargetOn [order 2] : [HandInTarget[targetA_row]==0]
    StayAtFirstTarget -> Show2ndTarget [order 1] : after(tickCount, e_clk)/
        | e_ApplyNewRotation
        | // apply the new rotation amount now (i.e. wait until the subject is in the starting target before applying a new
        | // rotation, so that they do not see the hand feedback jump/change when a new rotation is applied)
        | // have this event occur on this transition, rather than in the "StayAtFirstTarget" state to ensure that the subject
        | // is really starting the trial.  Could have put this event in the "Show2ndTarget" state instead.
    Show2ndTarget -> StayAt2ndTarget [order 2] : [HandInTarget[targetB_row]==1]
    Show2ndTarget -> EndOfTrial [order 1] : after(tickCount, e_clk)/
    StayAt2ndTarget -> EndOfTrial : after(tickCount, e_clk)
  state Initialize/
    // Turn off both targets, set hand_feedback on
    targetA_state=0;
    targetB_state=0;
  state Inter_Trial_State/
    // send e_Trial_End event
    e_Trial_End;
    // turn off both targets
    // stop data logging
    event_code=0;
    targetA_state=0;
    targetB_state=0;
    logging_enable = 0;
  (default) -> Initialize
  Initialize -> FirstTargetOn
  Inter_Trial_State -> FirstTargetOn : after(tickCount, e_clk)
  Main_Trial -> Inter_Trial_State : e_ExitTrialNow/
      | // if e_ExitTrialNow event occurs...
      | tickCount=1;
  EndOfTrial -> Inter_Trial_State
  data: logging_enable output boolean; event_code output uint16 [0..] =0; Trial_Protocol input double; HandInTarget input double; targetA_row output [1..32]; targetA_state output double; targetB_row output double; targetB_state output double; tickCount local double; load_row output double; reach_state output double; duration output double
  data targetA_row settings: description=index of the row currently being used in the TargetTable
  events: e_ApplyNewRotation output EITHER_EDGE_EVENT; e_clk input RISING_EDGE_EVENT; e_ExitTrialNow input EITHER_EDGE_EVENT; e_Trial_End output EITHER_EDGE_EVENT; e_start output EITHER_EDGE_EVENT

== matlab function vrm_plus_ff_return_backup/Visual_Rotation/Triggered Subsystem/Embedded MATLAB Function ==
  settings: fimath=|
      | fimath(...
      | 'RoundMode', 'floor',...
      | 'OverflowMode', 'wrap',...
      | 'ProductMode', 'KeepLSB', 'ProductWordLength', 32,...
      | 'SumMode', 'KeepLSB', 'SumWordLength', 32,...
      | 'CastBeforeSum', false)
  data: rotation output; Trial_Protocol input
function rotation   = Calculate_Desired_Rotation(Trial_Protocol)
% This block supports an embeddable subset of the MATLAB language.
% See the help menu for details. 

%This block was modified by IEB, Sept 24, 2008
%It updates the desired amount of rotation

% NOTE ALL ROTATIONS ARE CURRENTLY IN DEGREES IN THE FUNCTION

% create a persistent variable to remember the rotation amount from one time-step to the next
persistent rotation_memory

if isempty(rotation_memory),            rotation_memory = 0;										end

% where to look in the TP table for these parameters
rotate_type_COL = 8;
rotation_amount_COL = 9;

rotate_type = Trial_Protocol(rotate_type_COL);
rotation_amount = Trial_Protocol(rotation_amount_COL);

if rotate_type == 0
	%set the rotation = 0
	rotation = 0;
elseif rotate_type ==1
	%set the rotation = specified amount
	rotation = rotation_amount;
elseif rotate_type == 2
	%set the rotation to change by specified amount
	rotation = rotation_memory + rotation_amount;
else
	%do nothing
	rotation = rotation_memory;
end

% save the rotation amount for the next time-step
rotation_memory = rotation;

== matlab function vrm_plus_ff_return_backup/Visual_Rotation/Embedded MATLAB Function ==
  settings: fimath=|
      | fimath(...
      | 'RoundMode', 'floor',...
      | 'OverflowMode', 'wrap',...
      | 'ProductMode', 'KeepLSB', 'ProductWordLength', 32,...
      | 'SumMode', 'KeepLSB', 'SumWordLength', 32,...
      | 'CastBeforeSum', false)
  data: VCODES output; rotation input; Trial_Protocol input; Target_Table input; CursorPos output; VCODES_IN input
function [VCODES, CursorPos]  = Rotation(rotation, Trial_Protocol, Target_Table, VCODES_IN)
% This block supports an embeddable subset of the MATLAB language.
% See the help menu for details. 

%This block was modified by IEB, Sept 24, 2008
%It rotates the cursor position around a location specified as a target in the Trial_Protocol.

% VCODEs are length VCODE_LENGTH.
% All dimensions are units of (m).
% VCODE index definition: 1-5 as the same for all target types
% 1 - Target type
%		1=circle
%		2=ellipse
%       3=rectangle
%		4=line
%       5=triangle
%		6 and higher - not implemented yet
% 2 - status
%		0=off
%		1=on
% 3 - x position (m)
% 4 - y position (m)

% column in target table to find the target to rotation about
rotation_center_COL = 3;

rotation_center_target = Trial_Protocol(rotation_center_COL);
x_center = Target_Table(rotation_center_target, 1) * 0.01;		%convert to meters
y_center = Target_Table(rotation_center_target, 2) * 0.01;		%convert to meters

rotation = rotation*pi/180;		%convert desired rotation from degrees to radians

VCODES = VCODES_IN;
CursorPos = VCODES(1:2,3:4);
T = [x_center, y_center; x_center, y_center];                       %translation matrix
R = [cos(rotation) -sin(rotation); sin(rotation) cos(rotation)];	%rotation matrix

CursorPos = CursorPos - T;				%translate
CursorPos = (R*CursorPos')';			%rotate
CursorPos = CursorPos + T;				%re-translate

VCODES(1:2,3:4) = CursorPos;			%apply updated positions back into the VCODEs
